simulink model "clik_jacobian_transpose"  (R2023a)
settings: Solver=VariableStepAuto  StartTime=0.0  StopTime=24*5  RelTol=1e-3
undefined symbols (not defined in the file or in its folder): DiscIntNeverNeededParam, K_trasp, q0, Tc
settings Model: Creator=Valentina Giannotti  LastModifiedBy=salpi
settings OptimizationCC: ReuseModelBlockBuffer=off

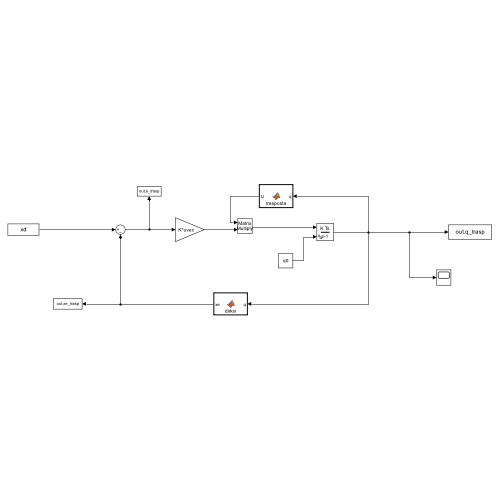
[thumbnail: Simulink's stored preview of the top-level diagram]
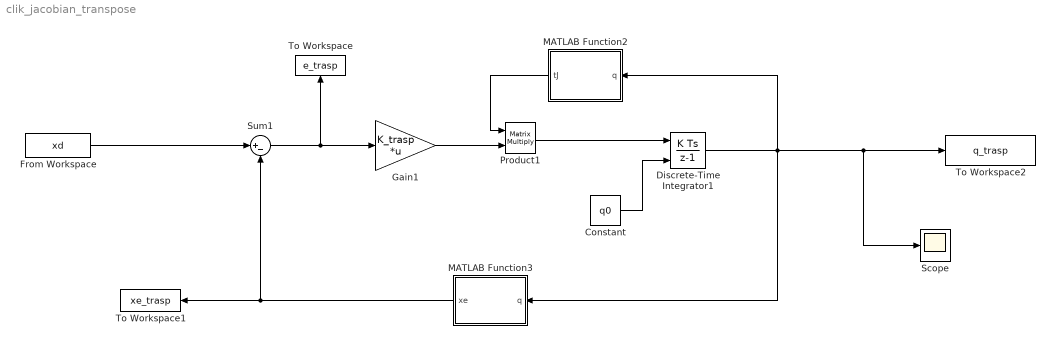
== system clik_jacobian_transpose ==
  Constant : Constant  Value=q0
  Discrete-Time Integrator1 : DiscreteIntegrator  InitialConditionSource=external  InitialCondition=[0 -pi/2 -0.5 pi/2]'  SampleTime=Tc  ICPrevOutput=DiscIntNeverNeededParam  ICPrevScaledInput=DiscIntNeverNeededParam
  From Workspace : FromWorkspace  VariableName=xd  SampleTime=Tc
  Gain1 : Gain  Gain=K_trasp  Multiplication=Matrix(K*u) (u vector)
  MATLAB Function2 : MATLAB Function  TreatAsAtomicUnit=on
  MATLAB Function3 : MATLAB Function  TreatAsAtomicUnit=on
  Product1 : Product  Multiplication=Matrix(*)
  Scope : Scope
  Sum1 : Sum  Inputs=|+-
  To Workspace : ToWorkspace  VariableName=e_trasp  SaveFormat=Structure With Time  SampleTime=-1
  To Workspace1 : ToWorkspace  VariableName=xe_trasp  SaveFormat=Structure With Time  SampleTime=-1
  To Workspace2 : ToWorkspace  VariableName=q_trasp  SaveFormat=Structure With Time  SampleTime=-1
  wires:
  Sum1/1 -> To Workspace/1, Gain1/1
  Constant/1 -> Discrete-Time Integrator1/2
  Product1/1 -> Discrete-Time Integrator1/1
  Gain1/1 -> Product1/2
  Discrete-Time Integrator1/1 -> MATLAB Function2/1(q), Scope/1, To Workspace2/1, MATLAB Function3/1(q)
  MATLAB Function2/1(tJ) -> Product1/1
  MATLAB Function3/1(xe) -> Sum1/2, To Workspace1/1
  From Workspace/1 -> Sum1/1

== matlab function clik_jacobian_transpose/MATLAB Function3 ==
  data: q input; xe output
function xe = dirkin(q)
% Pose in base coordinates, ordered as [x; y; z; phi].
a1=0.5;
a2=a1;
d0=1;

xe=[a1*cos(q(1))+a2*cos(q(1)+q(2));...
    a1*sin(q(1))+a2*sin(q(1)+q(2));...
    d0+q(3);...
    q(1)+q(2)+q(4)];
end

== matlab function clik_jacobian_transpose/MATLAB Function2 ==
  data: tJ output; q input
function tJ=trasposta(q)
% The transpose maps pose error to a joint-space correction.
a1=0.5;
a2=a1;

J=[-a1*sin(q(1))-a2*sin(q(1)+q(2)),-a2*sin(q(1)+q(2)),0,0;...
    a1*cos(q(1))+a2*cos(q(1)+q(2)),a2*cos(q(1)+q(2)),0,0;...
    0,0,1,0;...
    1,1,0,1];
tJ=J';
end
